simulink model "day3"  (R2024a)
settings: Solver=ode45  StartTime=0.0  StopTime=4  RelTol=1e-9  AbsTol=1e-11
settings Model: Creator=user  LastModifiedBy=user

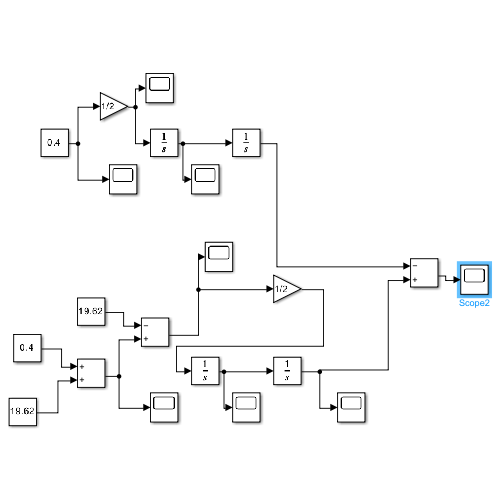
[thumbnail: Simulink's stored preview of the top-level diagram]
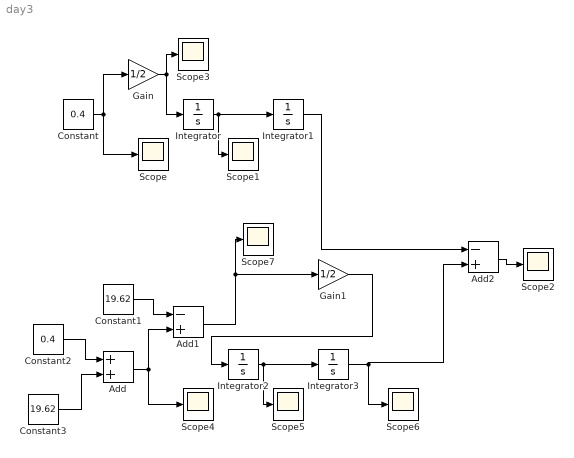
== system day3 ==
  Add : Sum
  Add1 : Sum  Inputs=-+
  Add2 : Sum  Inputs=-+
  Constant : Constant  Value=0.4  SampleTime=0.002
  Constant1 : Constant  Value=19.62  SampleTime=0.01
  Constant2 : Constant  Value=0.4  SampleTime=0.01
  Constant3 : Constant  Value=19.62  SampleTime=0.01
  Gain : Gain  Gain=1/2
  Gain1 : Gain  Gain=1/2
  Integrator : Integrator  ContinuousStateAttributes="\"velocity\""
  Integrator1 : Integrator  ContinuousStateAttributes="\"altitude\""
  Integrator2 : Integrator  ContinuousStateAttributes="\"velocity\""
  Integrator3 : Integrator  ContinuousStateAttributes="\"altitude\""
  Scope{,1..7} (8 alike) : Scope
  wires:
  Constant/1 -> Scope/1, Gain/1
  Integrator/1 -> Scope1/1, Integrator1/1
  Integrator1/1 -> Add2/1
  Gain/1 -> Integrator/1, Scope3/1
  Add1/1 -> Gain1/1, Scope7/1
  Integrator2/1 -> Scope5/1, Integrator3/1
  Integrator3/1 -> Scope6/1, Add2/2
  Add/1 -> Add1/2, Scope4/1
  Constant2/1 -> Add/1
  Constant3/1 -> Add/2
  Constant1/1 -> Add1/1
  Gain1/1 -> Integrator2/1
  Add2/1 -> Scope2/1
